simulink model "EV_Bus_Forward_before_compensation"  (R2025a)
settings: Solver=ode23t  StartTime=0.0  StopTime=300  MaxStep=0.01  RelTol=1e-5  AbsTol=1e-7
model workspace (MAT data in the model file):
  P.Mass = 20000
  P.Gravity = 9.81
  P.MotorCount = 2
  P.MotorPower = 400000
  P.MotorPeakTorque = 2500
  P.RegenPeakTorque = 1500
  P.RegenPower = 250000
  P.MaxRPM = 12000
  P.GearRatio = 21
  P.GearEfficiency = 0.97
  P.WheelRadius = 0.5
  P.Cd = 0.65
  P.FrontalArea = 8
  P.Crr = 0.008
  P.AirPressure = 101325
  P.AirGasConstant = 287.05
  P.MotorLag = 0.05
  P.BrakeLag = 0.25
  P.BrakeDelay = 0.1
  P.MaxBrakeTorque = 60000
  P.MaxPressure = 8
  P.DriverKp = 0.22
  P.DriverKi = 0.035
  P.DriverKaw = 2
  P.RegenFadeSpeed = 2
  P.RollingFadeSpeed = 0.2
  SignalNames = {'Environment_DesiredSpeed_kmph'; 'Environment_RoadSlope_pct'; 'Environment_AmbientTemp_degC'; 'Driver_Accelerator_pct'; 'Driver_Brake_pct'; 'Powertrain_Controller_MotorCommandTotal_Nm'; 'Powertrain_Controller_BrakeDemandWheel_Nm'; 'Electric_Drive_ActualMotorTotal_Nm'; 'Electric_Drive_ActualMotorEach_Nm'; 'Electric_Drive_ActualMotorSpeed_rpm'; 'Electric_Drive_MechanicalPower_kW'; 'Final_Drive_WheelDriveTorque_Nm'; 'Final_Drive_MotorSpeed_rpm'; 'Final_Drive_FinalDriveRatio'; 'Vehicle_Dynamics_VehicleSpeed_mps'; 'Vehicle_Dynamics_VehicleSpeed_kmph'; 'Vehicle_Dynamics_Acceleration_mps2'; 'Vehicle_Dynamics_AccelerationForce_N'; 'Vehicle_Dynamics_GradientForce_N'; 'Vehicle_Dynamics_RollingResistanceForce_N'; 'Vehicle_Dynamics_AerodynamicForce_N'; 'Vehicle_Dynamics_WheelTractionForce_N'; 'Vehicle_Dynamics_DriveForce_N'; 'Vehicle_Dynamics_FrictionBrakeForce_N'; 'Vehicle_Dynamics_StandstillReaction_N'; 'Vehicle_Dynamics_Distance_m'; 'Pneumatic_Brake_FrictionBrakeTorque_Nm'; 'Pneumatic_Brake_ChamberPressure_bar'}
  SlopeProfile = [0  0; 85  0; 100  4; 140  4; 155  0; 180  -3; 200  0; 300  0]
  SpeedProfile = [0  0; 5  0; 25  40; 55  40; 70  0; 85  0; 105  60; 140  60; 160  40; 180  40; 200  0; 225  0; 245  50; 260  50; 280  0; 300  0]
  TemperatureProfile = [0  25; 150  30; 300  35]
values from neighbouring files (symbols this model uses):
  P =     [EV_Bus_parameters.mat]
settings Model: Creator=Karuna  LastModifiedBy=Karuna
settings DataIOCC: SignalLogging=off  ReturnWorkspaceOutputs=off

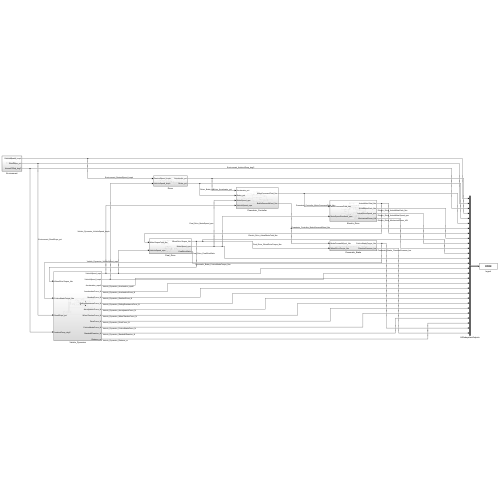
[thumbnail: Simulink's stored preview of the top-level diagram]
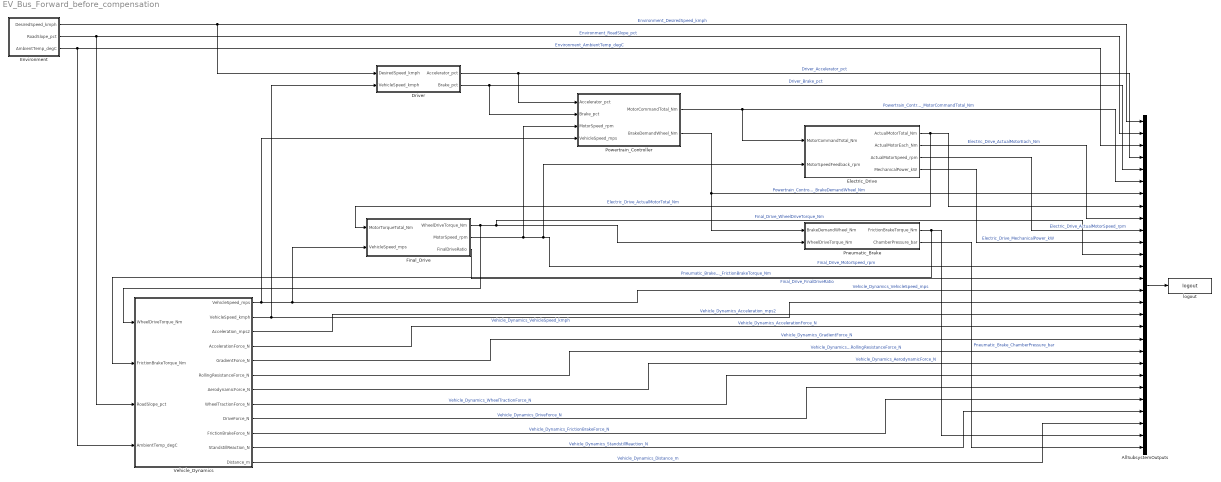
== system EV_Bus_Forward_before_compensation ==
  AllSubsystemOutputs : BusCreator  Inputs=28
  Driver : Subsystem  Description=PI speed driver with saturation feedback and integral limits. Non-overlapping accelerator and brake pedals, 0-100%. Minimum 15% holding brake when target <=0.1 km/h.
  Electric_Drive : Subsystem  Description=Equivalent combined model of two identical motors sharing torque equally at common speed. 50 ms torque response; actual torque limited to combined 800 kW drive / 500 kW regen and 5000 / -3000 Nm. Electrical supply assumed available; SOC and thermal dynamics omitted.
  Environment : Subsystem  Description=Linearly interpolated synthetic drive cycle, grade (%) and ambient temperature (degC). Edit SpeedProfile, SlopeProfile and TemperatureProfile in the model workspace.
  Final_Drive : Subsystem  Description=Fixed 21:1 reduction, 0.5 m wheel radius, 97% efficiency. Driving wheel torque = motor torque*21*0.97; regenerative wheel torque = motor torque*21/0.97. RPM comes from actual vehicle speed (no tire slip).
  Pneumatic_Brake : Subsystem  Description=Residual wheel brake demand after actual regenerative torque. Pressure proportional to request, 0.10 s air-line delay and 0.25 s first-order chamber response. 8 bar corresponds to total wheel friction torque 60000 Nm. Reduced-order pneumatic model.
  Powertrain_Controller : Subsystem  Description=Combined command for two equal 400 kW motors. Positive = driving; negative = regeneration. Torque/power envelope, overspeed traction inhibition and regen fade below 2 m/s. Service braking demand is total wheel torque.
  Vehicle_Dynamics : Subsystem  Description=Forward longitudinal dynamics: acceleration from net wheel force / 20000 kg, integrated into speed. Grade=atan(percent/100). Temperature changes air density. Traction = acceleration+gradient+rolling+aerodynamic forces. Forward-only standstill constraint reaction is separately logged. No tire slip, reverse or rotational inertia.
  logout : ToWorkspace  VariableName=logout  SaveFormat=Structure With Time  SampleTime=0.01
  wires:
  AllSubsystemOutputs/1 -> logout/1
  Pneumatic_Brake/2(ChamberPressure_bar) -> AllSubsystemOutputs/28  "Pneumatic_Brake_ChamberPressure_bar"
  Vehicle_Dynamics/12(Distance_m) -> AllSubsystemOutputs/26  "Vehicle_Dynamics_Distance_m"
  Vehicle_Dynamics/11(StandstillReaction_N) -> AllSubsystemOutputs/25  "Vehicle_Dynamics_StandstillReaction_N"
  Vehicle_Dynamics/10(FrictionBrakeForce_N) -> AllSubsystemOutputs/24  "Vehicle_Dynamics_FrictionBrakeForce_N"
  Vehicle_Dynamics/9(DriveForce_N) -> AllSubsystemOutputs/23  "Vehicle_Dynamics_DriveForce_N"
  Vehicle_Dynamics/8(WheelTractionForce_N) -> AllSubsystemOutputs/22  "Vehicle_Dynamics_WheelTractionForce_N"
  Vehicle_Dynamics/7(AerodynamicForce_N) -> AllSubsystemOutputs/21  "Vehicle_Dynamics_AerodynamicForce_N"
  Vehicle_Dynamics/6(RollingResistanceForce_N) -> AllSubsystemOutputs/20  "Vehicle_Dynamics_RollingResistanceForce_N"
  Vehicle_Dynamics/5(GradientForce_N) -> AllSubsystemOutputs/19  "Vehicle_Dynamics_GradientForce_N"
  Vehicle_Dynamics/4(AccelerationForce_N) -> AllSubsystemOutputs/18  "Vehicle_Dynamics_AccelerationForce_N"
  Vehicle_Dynamics/3(Acceleration_mps2) -> AllSubsystemOutputs/17  "Vehicle_Dynamics_Acceleration_mps2"
  Final_Drive/3(FinalDriveRatio) -> AllSubsystemOutputs/14  "Final_Drive_FinalDriveRatio"
  Electric_Drive/4(MechanicalPower_kW) -> AllSubsystemOutputs/11  "Electric_Drive_MechanicalPower_kW"
  Electric_Drive/3(ActualMotorSpeed_rpm) -> AllSubsystemOutputs/10  "Electric_Drive_ActualMotorSpeed_rpm"
  Electric_Drive/2(ActualMotorEach_Nm) -> AllSubsystemOutputs/9  "Electric_Drive_ActualMotorEach_Nm"
  Powertrain_Controller/2(BrakeDemandWheel_Nm) -> Pneumatic_Brake/1(BrakeDemandWheel_Nm), AllSubsystemOutputs/7  "Powertrain_Controller_BrakeDemandWheel_Nm"
  Environment/3(AmbientTemp_degC) -> AllSubsystemOutputs/3, Vehicle_Dynamics/4(AmbientTemp_degC)  "Environment_AmbientTemp_degC"
  Environment/2(RoadSlope_pct) -> Vehicle_Dynamics/3(RoadSlope_pct), AllSubsystemOutputs/2  "Environment_RoadSlope_pct"
  Pneumatic_Brake/1(FrictionBrakeTorque_Nm) -> Vehicle_Dynamics/2(FrictionBrakeTorque_Nm), AllSubsystemOutputs/27  "Pneumatic_Brake_FrictionBrakeTorque_Nm"
  Final_Drive/1(WheelDriveTorque_Nm) -> Pneumatic_Brake/2(WheelDriveTorque_Nm), AllSubsystemOutputs/12, Vehicle_Dynamics/1(WheelDriveTorque_Nm)  "Final_Drive_WheelDriveTorque_Nm"
  Electric_Drive/1(ActualMotorTotal_Nm) -> Final_Drive/1(MotorTorqueTotal_Nm), AllSubsystemOutputs/8  "Electric_Drive_ActualMotorTotal_Nm"
  Powertrain_Controller/1(MotorCommandTotal_Nm) -> Electric_Drive/1(MotorCommandTotal_Nm), AllSubsystemOutputs/6  "Powertrain_Controller_MotorCommandTotal_Nm"
  Vehicle_Dynamics/1(VehicleSpeed_mps) -> Final_Drive/2(VehicleSpeed_mps), AllSubsystemOutputs/15, Powertrain_Controller/4(VehicleSpeed_mps)  "Vehicle_Dynamics_VehicleSpeed_mps"
  Final_Drive/2(MotorSpeed_rpm) -> Electric_Drive/2(MotorSpeedFeedback_rpm), AllSubsystemOutputs/13, Powertrain_Controller/3(MotorSpeed_rpm)  "Final_Drive_MotorSpeed_rpm"
  Driver/2(Brake_pct) -> Powertrain_Controller/2(Brake_pct), AllSubsystemOutputs/5  "Driver_Brake_pct"
  Driver/1(Accelerator_pct) -> Powertrain_Controller/1(Accelerator_pct), AllSubsystemOutputs/4  "Driver_Accelerator_pct"
  Vehicle_Dynamics/2(VehicleSpeed_kmph) -> Driver/2(VehicleSpeed_kmph), AllSubsystemOutputs/16  "Vehicle_Dynamics_VehicleSpeed_kmph"
  Environment/1(DesiredSpeed_kmph) -> Driver/1(DesiredSpeed_kmph), AllSubsystemOutputs/1  "Environment_DesiredSpeed_kmph"

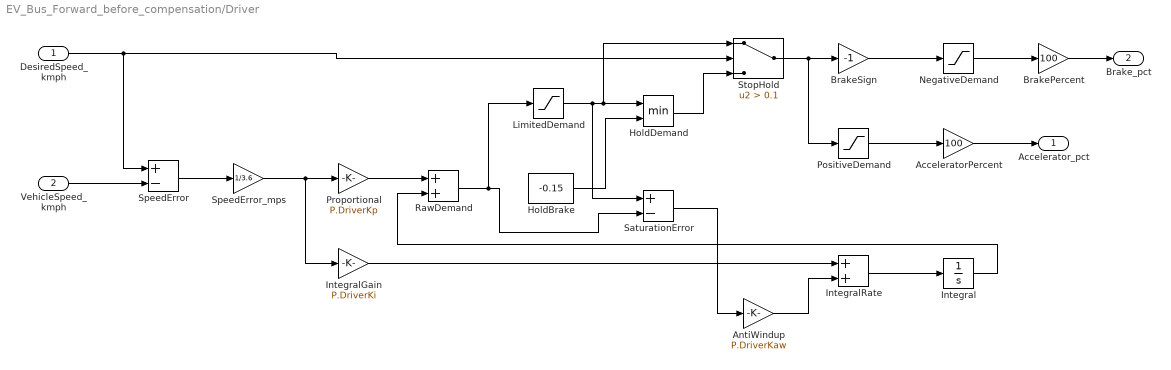
== system EV_Bus_Forward_before_compensation/Driver ==
  DesiredSpeed_kmph : Inport
  VehicleSpeed_kmph : Inport  Port=2
  AcceleratorPercent : Gain  Gain=100
  AntiWindup : Gain  Gain=P.DriverKaw
  BrakePercent : Gain  Gain=100
  BrakeSign : Gain  Gain=-1
  HoldBrake : Constant  Value=-0.15
  HoldDemand : MinMax  Inputs=2
  Integral : Integrator  LimitOutput=on  UpperSaturationLimit=0.6  LowerSaturationLimit=-0.6
  IntegralGain : Gain  Gain=P.DriverKi
  IntegralRate : Sum
  LimitedDemand : Saturate  UpperLimit=1  LowerLimit=-1
  NegativeDemand : Saturate  UpperLimit=1  LowerLimit=0
  PositiveDemand : Saturate  UpperLimit=1  LowerLimit=0
  Proportional : Gain  Gain=P.DriverKp
  RawDemand : Sum
  SaturationError : Sum  Inputs=+-
  SpeedError : Sum  Inputs=+-
  SpeedError_mps : Gain  Gain=1/3.6
  StopHold : Switch  Criteria=u2 > Threshold  Threshold=0.1  SaturateOnIntegerOverflow=off  InputSameDT=off
  Accelerator_pct : Outport
  Brake_pct : Outport  Port=2
  wires:
  BrakePercent/1 -> Brake_pct/1
  NegativeDemand/1 -> BrakePercent/1
  BrakeSign/1 -> NegativeDemand/1
  AcceleratorPercent/1 -> Accelerator_pct/1
  PositiveDemand/1 -> AcceleratorPercent/1
  StopHold/1 -> PositiveDemand/1, BrakeSign/1
  HoldDemand/1 -> StopHold/3
  HoldBrake/1 -> HoldDemand/2
  IntegralRate/1 -> Integral/1
  AntiWindup/1 -> IntegralRate/2
  IntegralGain/1 -> IntegralRate/1
  SaturationError/1 -> AntiWindup/1
  LimitedDemand/1 -> HoldDemand/1, StopHold/1, SaturationError/1
  RawDemand/1 -> LimitedDemand/1, SaturationError/2
  Integral/1 -> RawDemand/2
  Proportional/1 -> RawDemand/1
  SpeedError_mps/1 -> Proportional/1, IntegralGain/1
  SpeedError/1 -> SpeedError_mps/1
  VehicleSpeed_kmph/1 -> SpeedError/2
  DesiredSpeed_kmph/1 -> SpeedError/1, StopHold/2

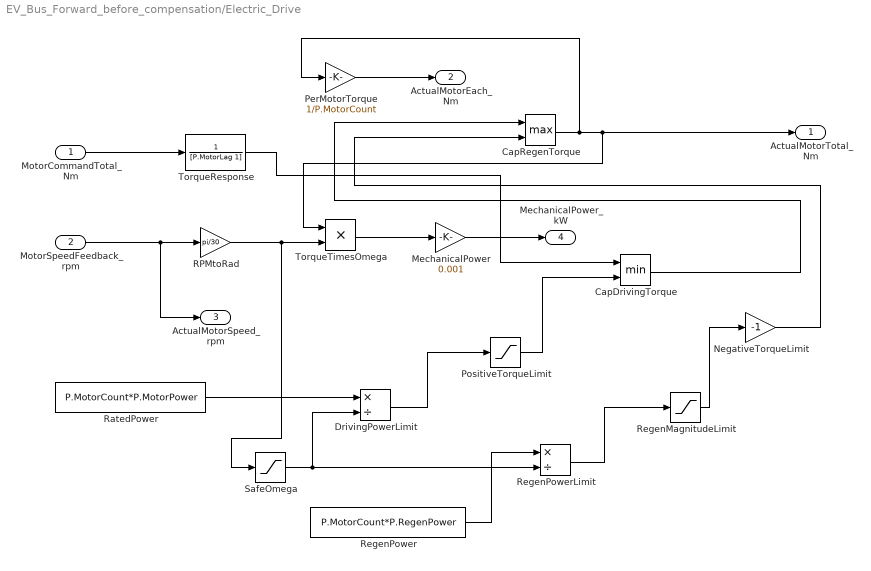
== system EV_Bus_Forward_before_compensation/Electric_Drive ==
  MotorCommandTotal_Nm : Inport
  MotorSpeedFeedback_rpm : Inport  Port=2
  CapDrivingTorque : MinMax  Inputs=2
  CapRegenTorque : MinMax  Function=max  Inputs=2
  DrivingPowerLimit : Product  Inputs=*/
  MechanicalPower : Gain  Gain=0.001
  NegativeTorqueLimit : Gain  Gain=-1
  PerMotorTorque : Gain  Gain=1/P.MotorCount
  PositiveTorqueLimit : Saturate  UpperLimit=P.MotorCount*P.MotorPeakTorque  LowerLimit=0
  RPMtoRad : Gain  Gain=pi/30
  RatedPower : Constant  Value=P.MotorCount*P.MotorPower
  RegenMagnitudeLimit : Saturate  UpperLimit=P.MotorCount*P.RegenPeakTorque  LowerLimit=0
  RegenPower : Constant  Value=P.MotorCount*P.RegenPower
  RegenPowerLimit : Product  Inputs=*/
  SafeOmega : Saturate  UpperLimit=inf  LowerLimit=1
  TorqueResponse : TransferFcn  Denominator=[P.MotorLag 1]
  TorqueTimesOmega : Product  Inputs=**
  ActualMotorTotal_Nm : Outport
  ActualMotorEach_Nm : Outport  Port=2
  ActualMotorSpeed_rpm : Outport  Port=3
  MechanicalPower_kW : Outport  Port=4
  wires:
  MechanicalPower/1 -> MechanicalPower_kW/1
  TorqueTimesOmega/1 -> MechanicalPower/1
  MotorSpeedFeedback_rpm/1 -> ActualMotorSpeed_rpm/1, RPMtoRad/1
  PerMotorTorque/1 -> ActualMotorEach_Nm/1
  MotorCommandTotal_Nm/1 -> TorqueResponse/1
  CapRegenTorque/1 -> TorqueTimesOmega/1, ActualMotorTotal_Nm/1, PerMotorTorque/1
  NegativeTorqueLimit/1 -> CapRegenTorque/2
  CapDrivingTorque/1 -> CapRegenTorque/1
  PositiveTorqueLimit/1 -> CapDrivingTorque/2
  RegenMagnitudeLimit/1 -> NegativeTorqueLimit/1
  RegenPowerLimit/1 -> RegenMagnitudeLimit/1
  RegenPower/1 -> RegenPowerLimit/1
  DrivingPowerLimit/1 -> PositiveTorqueLimit/1
  SafeOmega/1 -> RegenPowerLimit/2, DrivingPowerLimit/2
  RatedPower/1 -> DrivingPowerLimit/1
  TorqueResponse/1 -> CapDrivingTorque/1
  RPMtoRad/1 -> SafeOmega/1, TorqueTimesOmega/2

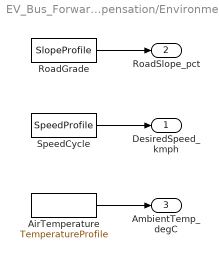
== system EV_Bus_Forward_before_compensation/Environment ==
  AirTemperature : FromWorkspace  VariableName=TemperatureProfile
  RoadGrade : FromWorkspace  VariableName=SlopeProfile
  SpeedCycle : FromWorkspace  VariableName=SpeedProfile
  DesiredSpeed_kmph : Outport
  RoadSlope_pct : Outport  Port=2
  AmbientTemp_degC : Outport  Port=3
  wires:
  AirTemperature/1 -> AmbientTemp_degC/1
  RoadGrade/1 -> RoadSlope_pct/1
  SpeedCycle/1 -> DesiredSpeed_kmph/1

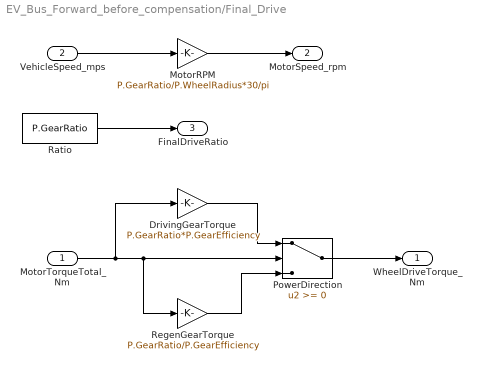
== system EV_Bus_Forward_before_compensation/Final_Drive ==
  MotorTorqueTotal_Nm : Inport
  VehicleSpeed_mps : Inport  Port=2
  DrivingGearTorque : Gain  Gain=P.GearRatio*P.GearEfficiency
  MotorRPM : Gain  Gain=P.GearRatio/P.WheelRadius*30/pi
  PowerDirection : Switch  SaturateOnIntegerOverflow=off  InputSameDT=off
  Ratio : Constant  Value=P.GearRatio
  RegenGearTorque : Gain  Gain=P.GearRatio/P.GearEfficiency
  WheelDriveTorque_Nm : Outport
  MotorSpeed_rpm : Outport  Port=2
  FinalDriveRatio : Outport  Port=3
  wires:
  Ratio/1 -> FinalDriveRatio/1
  MotorRPM/1 -> MotorSpeed_rpm/1
  VehicleSpeed_mps/1 -> MotorRPM/1
  PowerDirection/1 -> WheelDriveTorque_Nm/1
  RegenGearTorque/1 -> PowerDirection/3
  DrivingGearTorque/1 -> PowerDirection/1
  MotorTorqueTotal_Nm/1 -> PowerDirection/2, RegenGearTorque/1, DrivingGearTorque/1

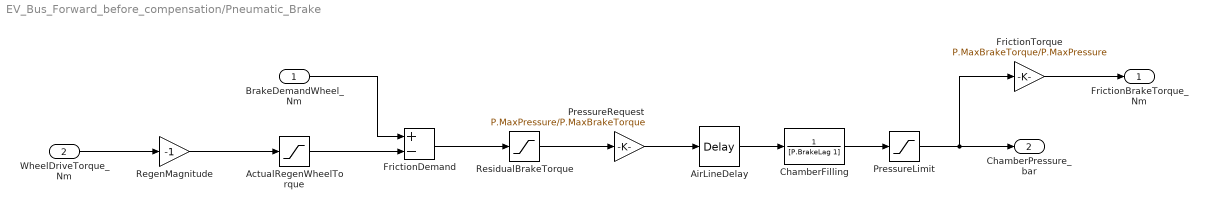
== system EV_Bus_Forward_before_compensation/Pneumatic_Brake ==
  BrakeDemandWheel_Nm : Inport
  WheelDriveTorque_Nm : Inport  Port=2
  ActualRegenWheelTorque : Saturate  UpperLimit=inf  LowerLimit=0
  AirLineDelay : TransportDelay  DelayTime=P.BrakeDelay
  ChamberFilling : TransferFcn  Denominator=[P.BrakeLag 1]
  FrictionDemand : Sum  Inputs=+-
  FrictionTorque : Gain  Gain=P.MaxBrakeTorque/P.MaxPressure
  PressureLimit : Saturate  UpperLimit=P.MaxPressure  LowerLimit=0
  PressureRequest : Gain  Gain=P.MaxPressure/P.MaxBrakeTorque
  RegenMagnitude : Gain  Gain=-1
  ResidualBrakeTorque : Saturate  UpperLimit=P.MaxBrakeTorque  LowerLimit=0
  FrictionBrakeTorque_Nm : Outport
  ChamberPressure_bar : Outport  Port=2
  wires:
  FrictionTorque/1 -> FrictionBrakeTorque_Nm/1
  PressureLimit/1 -> ChamberPressure_bar/1, FrictionTorque/1
  ChamberFilling/1 -> PressureLimit/1
  AirLineDelay/1 -> ChamberFilling/1
  PressureRequest/1 -> AirLineDelay/1
  ResidualBrakeTorque/1 -> PressureRequest/1
  FrictionDemand/1 -> ResidualBrakeTorque/1
  ActualRegenWheelTorque/1 -> FrictionDemand/2
  BrakeDemandWheel_Nm/1 -> FrictionDemand/1
  RegenMagnitude/1 -> ActualRegenWheelTorque/1
  WheelDriveTorque_Nm/1 -> RegenMagnitude/1

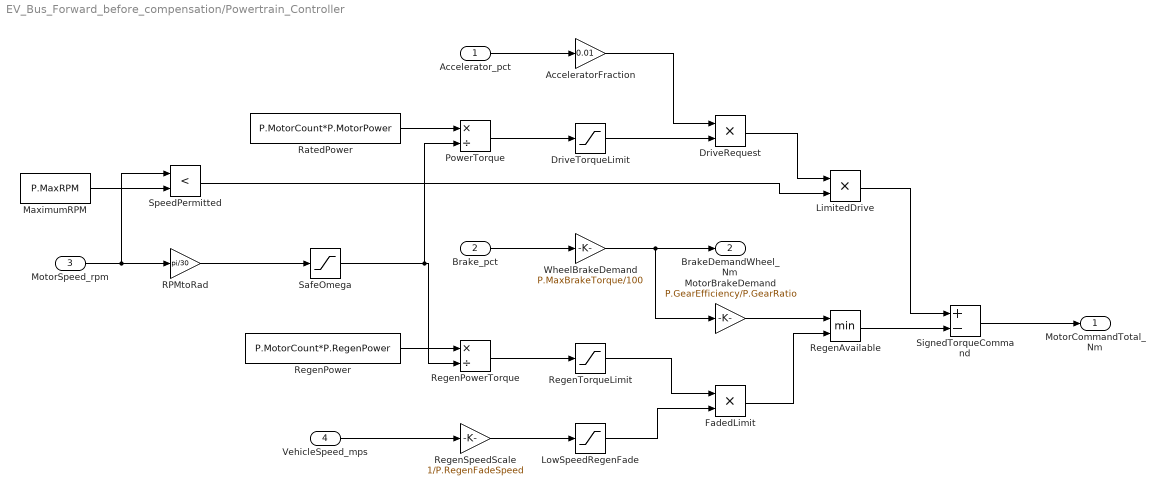
== system EV_Bus_Forward_before_compensation/Powertrain_Controller ==
  Accelerator_pct : Inport
  Brake_pct : Inport  Port=2
  MotorSpeed_rpm : Inport  Port=3
  VehicleSpeed_mps : Inport  Port=4
  AcceleratorFraction : Gain  Gain=0.01
  DriveRequest : Product  Inputs=**
  DriveTorqueLimit : Saturate  UpperLimit=P.MotorCount*P.MotorPeakTorque  LowerLimit=0
  FadedLimit : Product  Inputs=**
  LimitedDrive : Product  Inputs=**
  LowSpeedRegenFade : Saturate  UpperLimit=1  LowerLimit=0
  MaximumRPM : Constant  Value=P.MaxRPM
  MotorBrakeDemand : Gain  Gain=P.GearEfficiency/P.GearRatio
  PowerTorque : Product  Inputs=*/
  RPMtoRad : Gain  Gain=pi/30
  RatedPower : Constant  Value=P.MotorCount*P.MotorPower
  RegenAvailable : MinMax  Inputs=2
  RegenPower : Constant  Value=P.MotorCount*P.RegenPower
  RegenPowerTorque : Product  Inputs=*/
  RegenSpeedScale : Gain  Gain=1/P.RegenFadeSpeed
  RegenTorqueLimit : Saturate  UpperLimit=P.MotorCount*P.RegenPeakTorque  LowerLimit=0
  SafeOmega : Saturate  UpperLimit=inf  LowerLimit=1
  SignedTorqueCommand : Sum  Inputs=+-
  SpeedPermitted : RelationalOperator  Operator=<  OutDataTypeStr=boolean  RndMeth=Simplest  InputSameDT=off
  WheelBrakeDemand : Gain  Gain=P.MaxBrakeTorque/100
  MotorCommandTotal_Nm : Outport
  BrakeDemandWheel_Nm : Outport  Port=2
  wires:
  SignedTorqueCommand/1 -> MotorCommandTotal_Nm/1
  RegenAvailable/1 -> SignedTorqueCommand/2
  LimitedDrive/1 -> SignedTorqueCommand/1
  SpeedPermitted/1 -> LimitedDrive/2
  DriveRequest/1 -> LimitedDrive/1
  FadedLimit/1 -> RegenAvailable/2
  LowSpeedRegenFade/1 -> FadedLimit/2
  RegenTorqueLimit/1 -> FadedLimit/1
  MotorBrakeDemand/1 -> RegenAvailable/1
  WheelBrakeDemand/1 -> BrakeDemandWheel_Nm/1, MotorBrakeDemand/1
  Brake_pct/1 -> WheelBrakeDemand/1
  MaximumRPM/1 -> SpeedPermitted/2
  DriveTorqueLimit/1 -> DriveRequest/2
  AcceleratorFraction/1 -> DriveRequest/1
  Accelerator_pct/1 -> AcceleratorFraction/1
  RegenSpeedScale/1 -> LowSpeedRegenFade/1
  VehicleSpeed_mps/1 -> RegenSpeedScale/1
  RegenPowerTorque/1 -> RegenTorqueLimit/1
  RegenPower/1 -> RegenPowerTorque/1
  PowerTorque/1 -> DriveTorqueLimit/1
  SafeOmega/1 -> PowerTorque/2, RegenPowerTorque/2
  RatedPower/1 -> PowerTorque/1
  RPMtoRad/1 -> SafeOmega/1
  MotorSpeed_rpm/1 -> SpeedPermitted/1, RPMtoRad/1

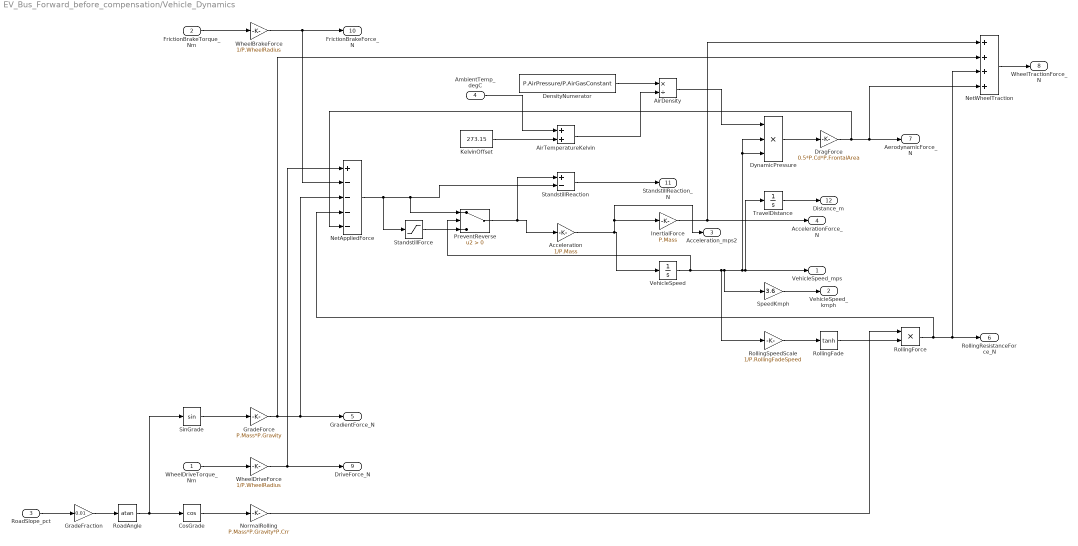
== system EV_Bus_Forward_before_compensation/Vehicle_Dynamics ==
  WheelDriveTorque_Nm : Inport
  FrictionBrakeTorque_Nm : Inport  Port=2
  RoadSlope_pct : Inport  Port=3
  AmbientTemp_degC : Inport  Port=4
  Acceleration : Gain  Gain=1/P.Mass
  AirDensity : Product  Inputs=*/
  AirTemperatureKelvin : Sum
  CosGrade : Trigonometry  Operator=cos
  DensityNumerator : Constant  Value=P.AirPressure/P.AirGasConstant
  DragForce : Gain  Gain=0.5*P.Cd*P.FrontalArea
  DynamicPressure : Product  Inputs=***
  GradeForce : Gain  Gain=P.Mass*P.Gravity
  GradeFraction : Gain  Gain=0.01
  InertialForce : Gain  Gain=P.Mass
  KelvinOffset : Constant  Value=273.15
  NetAppliedForce : Sum  Inputs=+----
  NetWheelTraction : Sum  Inputs=++++
  NormalRolling : Gain  Gain=P.Mass*P.Gravity*P.Crr
  PreventReverse : Switch  Criteria=u2 > Threshold  SaturateOnIntegerOverflow=off  InputSameDT=off
  RoadAngle : Trigonometry  Operator=atan
  RollingFade : Trigonometry  Operator=tanh
  RollingForce : Product  Inputs=**
  RollingSpeedScale : Gain  Gain=1/P.RollingFadeSpeed
  SinGrade : Trigonometry
  SpeedKmph : Gain  Gain=3.6
  StandstillForce : Saturate  UpperLimit=inf  LowerLimit=0
  StandstillReaction : Sum  Inputs=+-
  TravelDistance : Integrator
  VehicleSpeed : Integrator  LimitOutput=on  LowerSaturationLimit=0
  WheelBrakeForce : Gain  Gain=1/P.WheelRadius
  WheelDriveForce : Gain  Gain=1/P.WheelRadius
  VehicleSpeed_mps : Outport
  VehicleSpeed_kmph : Outport  Port=2
  Acceleration_mps2 : Outport  Port=3
  AccelerationForce_N : Outport  Port=4
  GradientForce_N : Outport  Port=5
  RollingResistanceForce_N : Outport  Port=6
  AerodynamicForce_N : Outport  Port=7
  WheelTractionForce_N : Outport  Port=8
  DriveForce_N : Outport  Port=9
  FrictionBrakeForce_N : Outport  Port=10
  StandstillReaction_N : Outport  Port=11
  Distance_m : Outport  Port=12
  wires:
  TravelDistance/1 -> Distance_m/1
  StandstillReaction/1 -> StandstillReaction_N/1
  NetWheelTraction/1 -> WheelTractionForce_N/1
  SpeedKmph/1 -> VehicleSpeed_kmph/1
  InertialForce/1 -> NetWheelTraction/1, AccelerationForce_N/1
  Acceleration/1 -> InertialForce/1, Acceleration_mps2/1, VehicleSpeed/1
  PreventReverse/1 -> Acceleration/1, StandstillReaction/1
  StandstillForce/1 -> PreventReverse/3
  NetAppliedForce/1 -> StandstillReaction/2, PreventReverse/1, StandstillForce/1
  DragForce/1 -> NetWheelTraction/4, AerodynamicForce_N/1, NetAppliedForce/5
  RollingForce/1 -> NetWheelTraction/3, RollingResistanceForce_N/1, NetAppliedForce/4
  GradeForce/1 -> NetAppliedForce/3, GradientForce_N/1, NetWheelTraction/2
  WheelBrakeForce/1 -> FrictionBrakeForce_N/1, NetAppliedForce/2
  WheelDriveForce/1 -> DriveForce_N/1, NetAppliedForce/1
  FrictionBrakeTorque_Nm/1 -> WheelBrakeForce/1
  WheelDriveTorque_Nm/1 -> WheelDriveForce/1
  DynamicPressure/1 -> DragForce/1
  AirDensity/1 -> DynamicPressure/1
  AirTemperatureKelvin/1 -> AirDensity/2
  DensityNumerator/1 -> AirDensity/1
  KelvinOffset/1 -> AirTemperatureKelvin/2
  AmbientTemp_degC/1 -> AirTemperatureKelvin/1
  RollingFade/1 -> RollingForce/2
  NormalRolling/1 -> RollingForce/1
  RollingSpeedScale/1 -> RollingFade/1
  VehicleSpeed/1 -> TravelDistance/1, VehicleSpeed_mps/1, DynamicPressure/2, DynamicPressure/3, SpeedKmph/1, RollingSpeedScale/1, PreventReverse/2
  CosGrade/1 -> NormalRolling/1
  SinGrade/1 -> GradeForce/1
  RoadAngle/1 -> SinGrade/1, CosGrade/1
  GradeFraction/1 -> RoadAngle/1
  RoadSlope_pct/1 -> GradeFraction/1
